simulink model "sf_slswitch"  (R2025b)
settings: Solver=ode45  StartTime=0.0  StopTime=10.0  MaxStep=.2  RelTol=1e-3  EnableMultiTasking=on
model workspace (MAT data in the model file):
  PID_TRESH = 0.3
undefined symbols (not defined in the file or in its folder): DiscIntNeverNeededParam
libraries: simulink x1
settings Model: Creator=The MathWorks, Inc.  LastModifiedBy=The MathWorks, Inc.
settings SolverCC: AlgebraicLoopSolver=TrustRegion
settings DataIOCC: LimitDataPoints=on  SaveFormat=Array  ReturnWorkspaceOutputs=off
settings OptimizationCC: ReuseModelBlockBuffer=off  ExpressionDepthLimit=2147483647.0  LifeSpan=inf
settings DebuggingCC: UnderspecifiedInitializationDetection=Classic  MergeDetectMultiDrivingBlocksExec=none  SolverPrmCheckMsg=warning  FcnCallInpInsideContextMsg=warning  UnconnectedInputMsg=warning  UnconnectedOutputMsg=warning  UnconnectedLineMsg=warning  StateNameClashWarn=warning  SFUnexpectedBacktrackingDiag=warning  SFNoUnconditionalDefaultTransitionDiag=warning  SFExecutionAtInitializationDiag=none  ArithmeticOperatorsInVariantConditions=warning
settings HardwareCC: ProdBitPerPointer=32.0  ProdBitPerSizeT=32.0  ProdBitPerPtrDiffT=32.0  ProdLargestAtomicFloat=None  ProdIntDivRoundTo=Undefined  ProdEndianess=Unspecified  ProdWordSize=32.0  ProdHWDeviceType=32-bit Generic
settings ModelReferenceCC: EnableRefExpFcnMdlSchedulingChecks=on  PropagateSignalLabelsOutOfModel=off
settings SFSimCC: SimUseLocalCustomCode=off  SimParseCustomCode=off  CustomCodeUndefinedFunction=UseInterfaceOnly
settings RTWCC: RTWUseLocalCustomCode=off  GPUComputeCapability=3.5
settings CodeAppCC: StateflowObjectComments=on
settings GRTTargetCC: TargetLangStandard=C89/C90 (ANSI)  CombineOutputUpdateFcns=off  GRTInterface=on
settings ConfigComp: CovMetricSettings=dw  CovSaveCumulativeToWorkspaceVar=on  CovSaveSingleToWorkspaceVar=on  CovExternalEMLEnable=off  CovSFcnEnable=off

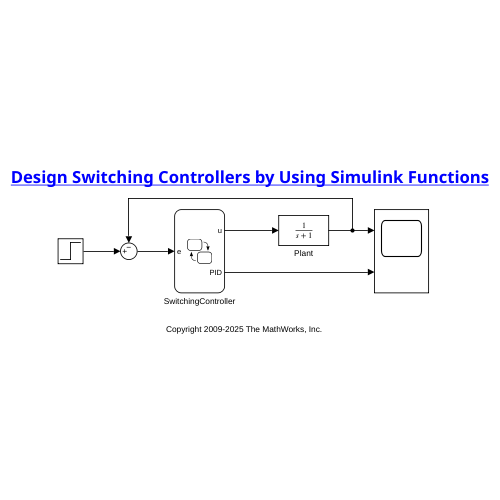
[thumbnail: Simulink's stored preview of the top-level diagram]
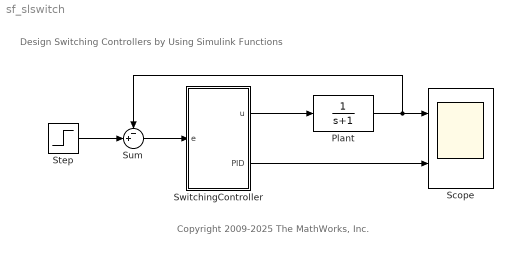
== system sf_slswitch ==
  note: Copyright 2009-2025 The MathWorks, Inc.
  note: Design Switching Controllers by Using Simulink Functions
  Plant : TransferFcn  Denominator=[1 1]
  Scope : Scope  NumInputPorts=2
      settings: ActiveDisplayYMinimum=0  ActiveDisplayYMaximum=1
  Step : Step  SampleTime=0
  Sum : Sum  Inputs=-+|
  SwitchingController : Stateflow chart  TreatAsAtomicUnit=on
  wires:
  Sum/1 -> SwitchingController/1(e)
  Plant/1 -> Sum/1, Scope/1
  SwitchingController/1(u) -> Plant/1
  Step/1 -> Sum/2
  SwitchingController/2(" PID") -> Scope/2

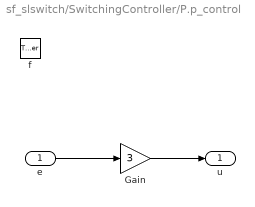
== system sf_slswitch/SwitchingController/P.p_control ==
  e : Inport
  f : TriggerPort  TriggerType=function-call  VariantControl=(inherit)
      settings: CopyFcn=Stateflow.SLINSF.SimulinkMan.removeBlockPreDeleteFcn  PreDeleteFcn=Stateflow.SLINSF.SimulinkMan.unsafePredeleteFcn
  Gain : Gain  Gain=3
  u : Outport  VectorParamsAs1DForOutWhenUnconnected=off
  wires:
  e/1 -> Gain/1
  Gain/1 -> u/1

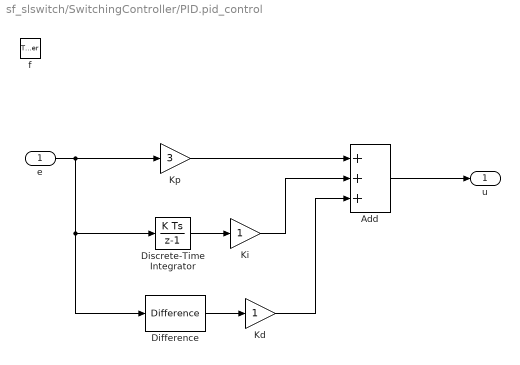
== system sf_slswitch/SwitchingController/PID.pid_control ==
  e : Inport
  f : TriggerPort  TriggerType=function-call  VariantControl=(inherit)
      settings: CopyFcn=Stateflow.SLINSF.SimulinkMan.removeBlockPreDeleteFcn  PreDeleteFcn=Stateflow.SLINSF.SimulinkMan.unsafePredeleteFcn
  Add : Sum  Inputs=+++
  Difference : simulink/Discrete/Difference  ICPrevInput=0.0  OutMin=[]  OutMax=[]  OutDataType=fixdt(1, 16)  OutScaling=2^-10  DoSatur=off
  Discrete-Time Integrator : DiscreteIntegrator  SampleTime=-1  ICPrevOutput=DiscIntNeverNeededParam  ICPrevScaledInput=DiscIntNeverNeededParam
  Kd : Gain
  Ki : Gain
  Kp : Gain  Gain=3
  u : Outport  VectorParamsAs1DForOutWhenUnconnected=off
  wires:
  e/1 -> Kp/1, Discrete-Time Integrator/1, Difference/1
  Kp/1 -> Add/1
  Add/1 -> u/1
  Discrete-Time Integrator/1 -> Ki/1
  Difference/1 -> Kd/1
  Ki/1 -> Add/2
  Kd/1 -> Add/3

== stateflow chart sf_slswitch/SwitchingController ==
  state STEADY
    entry: u = 0;
  state P
    du:
    u = p_control(e);
    state u = p_control(e) [function]
  state PID
    du:
    u = pid_control(e);
    state u = pid_control(e) [function]
  (default) -> STEADY
  P -> PID : [e < PID_TRESH]
  STEADY -> P : [e > 0.01]
  data: e function_input; u function_output; e function_input; u function_output; e input; u output double; PID output boolean; PID_TRESH parameter
